simulink model "MMC_21_Level_Rectifier"  (R2023b)
settings: Solver=FixedStepAuto  StartTime=0.0  StopTime=0.5  RelTol=1e-3
libraries: spsSeriesRLCBranchLib x71, spsVoltageMeasurementLib x69, spsUniversalBridgeLib x60, spsCurrentMeasurementLib x8, slpidlib x7, spsRMSLib x3, spsACVoltageSourceLib x3, spsMeanLib x2, simulink x1, spsTHDLib x1, spspowerguiLib x1
(part 1 of 4)
settings Model: SimulationMode=accelerator  Creator=abc6820292  LastModifiedBy=Qu
settings SolverCC: ZeroCrossAlgorithm=Adaptive
settings DataIOCC: ReturnWorkspaceOutputs=off  Refine=10
settings DebuggingCC: IgnoredZcDiagnostic=none  UnconnectedInputMsg=warning  UnconnectedOutputMsg=warning  UnconnectedLineMsg=warning
settings ModelReferenceCC: EnableRefExpFcnMdlSchedulingChecks=on
settings RTWCC: DLArmComputeVersion=19.05

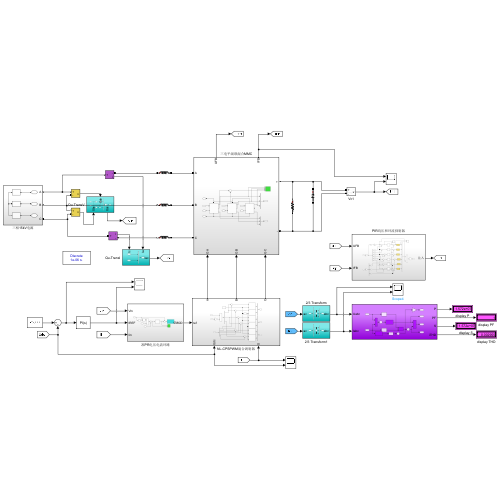
[thumbnail: Simulink's stored preview of the top-level diagram]
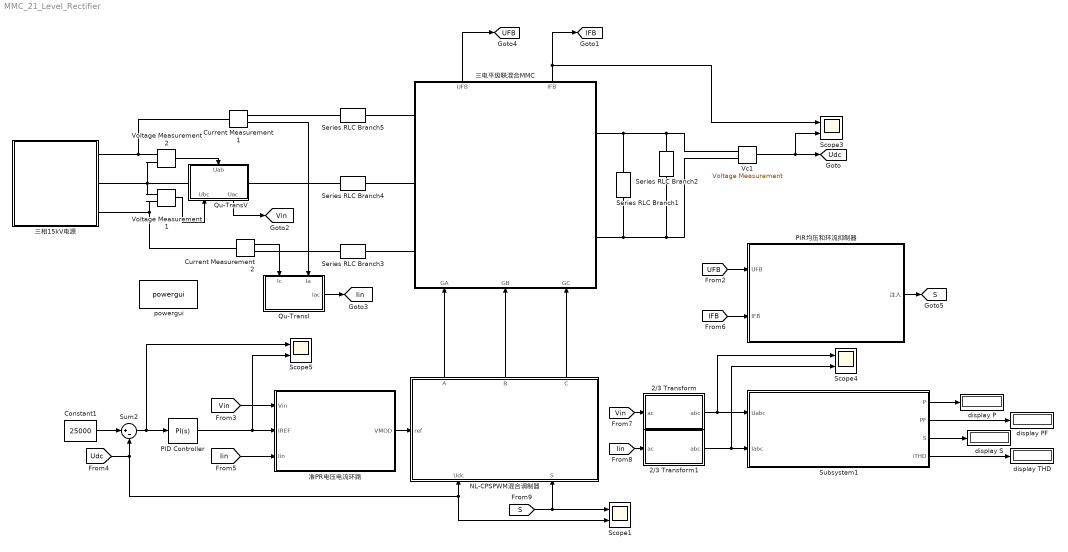
== system MMC_21_Level_Rectifier ==
  2/3 Transform : Subsystem
      settings: PortSchema="{\"entries\":[{\"content\":{\"sides\":[{\"content\":{},\"type\":\"ConnectorPlacement.EquallySpacedRectSide\",\"uuid\":\"58c40194-9a95-4e39-952e-f878bde7484e\"},{\"content\":{\"side\":\"RIGHT\"},\"type\":\"ConnectorPlacement.EquallySpacedRectSide\",\"uuid\":\"f51692e8-3ff2-4d72-808d-3667196a4526\"},{\"content\":{\"connectorIds\":[\"In1\"],\"side\":\"TOP\"},\"type\":\"ConnectorPlacement.EquallySpacedRectSide\",\"uuid\":\"0aab136b-5da5-45c4-8998-999ebe8b7f2f\"},{\"content\":{\"connectorIds\":[\"Out1\"],\"side\":\"BOTTOM\"},\"type\":\"ConnectorPlacement.EquallySpacedRectSide\",\"uuid\":\"32f5f4a5-4ebb-496b-828d-b973bd46b44e\"}]},\"type\":\"ConnectorPlacement.EquallySpacedConnector\",\"uuid\":\"3ef81af7-d426-47fb-88e3-e33e58eebb83\"}],\"packageUris\":[\"http://schema.mathworks.com/mf0/Connector/R2020b\"],\"version\":\"1.0\"}"
  2/3 Transform1 : Subsystem
      settings: PortSchema="{\"entries\":[{\"content\":{\"sides\":[{\"content\":{},\"type\":\"ConnectorPlacement.EquallySpacedRectSide\",\"uuid\":\"58c40194-9a95-4e39-952e-f878bde7484e\"},{\"content\":{\"side\":\"RIGHT\"},\"type\":\"ConnectorPlacement.EquallySpacedRectSide\",\"uuid\":\"f51692e8-3ff2-4d72-808d-3667196a4526\"},{\"content\":{\"connectorIds\":[\"In1\"],\"side\":\"TOP\"},\"type\":\"ConnectorPlacement.EquallySpacedRectSide\",\"uuid\":\"0aab136b-5da5-45c4-8998-999ebe8b7f2f\"},{\"content\":{\"connectorIds\":[\"Out1\"],\"side\":\"BOTTOM\"},\"type\":\"ConnectorPlacement.EquallySpacedRectSide\",\"uuid\":\"32f5f4a5-4ebb-496b-828d-b973bd46b44e\"}]},\"type\":\"ConnectorPlacement.EquallySpacedConnector\",\"uuid\":\"3ef81af7-d426-47fb-88e3-e33e58eebb83\"}],\"packageUris\":[\"http://schema.mathworks.com/mf0/Connector/R2020b\"],\"version\":\"1.0\"}"
  Constant1 : Constant  Value=25000
  Current Measurement1 : spsCurrentMeasurementLib/Current Measurement  PhasorSimulation=off  OutputType=Complex  PSBequivalent=0
  Current Measurement2 : spsCurrentMeasurementLib/Current Measurement  PhasorSimulation=off  OutputType=Complex  PSBequivalent=0
  NL-CPSPWM混合调制器 : Subsystem
      settings: PortSchema="{\"entries\":[{\"content\":{\"sides\":[{\"content\":{\"connectorIds\":[\"In1\"]},\"type\":\"ConnectorPlacement.EquallySpacedRectSide\",\"uuid\":\"86d8a801-af54-4615-919a-9a70996995f5\"},{\"content\":{\"side\":\"RIGHT\"},\"type\":\"ConnectorPlacement.EquallySpacedRectSide\",\"uuid\":\"9c099dd5-197a-4a29-8cd5-6822de601230\"},{\"content\":{\"connectorIds\":[\"Out1\",\"Out2\",\"Out3\"],\"side\":\"TOP\"},\"type\":\"ConnectorPlacement.EquallySpacedRectSide\",\"uuid\":\"5852d946-2383-4602-be71-32d16fa24bc3\"},{\"content\":{\"connectorIds\":[\"In2\",\"In3\"],\"side\":\"BOTTOM\"},\"type\":\"ConnectorPlacement.EquallySpacedRectSide\",\"uuid\":\"40763eea-52f3-43b7-92a8-ded335eb8a8b\"}]},\"type\":\"ConnectorPlacement.EquallySpacedConnector\",\"uuid\":\"a21c857f-e780-49b2-9a65-1676cf4540b1\"}],\"packageUris\":[\"http://schema.mathworks.com/mf0/Connector/R2020b\"],\"version\":\"1.0\"}"
  PID Controller : slpidlib/PID Controller  Controller=PI  Form=Parallel  TimeDomain=Continuous-time  UseExternalTs=off  SampleTime=-1  IntegratorMethod=Forward Euler  FilterMethod=Forward Euler  ControllerParametersSource=internal  P=0.12  I=6  UseKiTs=off  D=0  N=100  UseFilter=on  TunerSelectOption=Transfer Function Based (PID Tuner App)  InitialConditionSource=internal  InitialConditionForIntegrator=0  InitialConditionForFilter=0  DifferentiatorICPrevScaledInput=0  ExternalReset=none  TrackingMode=off  Kt=1  LimitOutput=off  SatLimitsSource=internal  UpperSaturationLimit=100  LowerSaturationLimit=-100  LinearizeAsGain=on  AntiWindupMode=none  Kb=1  LimitIntegrator=off  UpperIntegratorSaturationLimit=inf  LowerIntegratorSaturationLimit=-inf  POutMin=[]  POutMax=[]  IOutMin=[]  IOutMax=[]  DOutMin=[]  DOutMax=[]  NOutMin=[]  NOutMax=[]  SumOutMin=[]  SumOutMax=[]  SaturationOutMin=[]  SaturationOutMax=[]  PParamMin=[]  PParamMax=[]  IParamMin=[]  IParamMax=[]  DParamMin=[]  DParamMax=[]  NParamMin=[]  NParamMax=[]  KbParamMin=[]  KbParamMax=[]  KtParamMin=[]  KtParamMax=[]  KbOutMin=[]  KbOutMax=[]  KtOutMin=[]  KtOutMax=[]  IntegratorOutMin=[]  IntegratorOutMax=[]  FilterOutMin=[]  FilterOutMax=[]  SumI1OutMin=[]  SumI1OutMax=[]  SumI2OutMin=[]  SumI2OutMax=[]  SumI3OutMin=[]  SumI3OutMax=[]  SumI4OutMin=[]  SumI4OutMax=[]  SumDOutMin=[]  SumDOutMax=[]  DifferentiatorOutMin=[]  DifferentiatorOutMax=[]  FilterDiffOutCoefMin=[]  FilterDiffOutCoefMax=[]  ReciprocalOutMin=[]  ReciprocalOutMax=[]  SumDenOutMin=[]  SumDenOutMax=[]  SumNumOutMin=[]  SumNumOutMax=[]  DivideOutMin=[]  DivideOutMax=[]  UdiffTsProdOutMin=[]  UdiffTsProdOutMax=[]  NTsProdOutMin=[]  NTsProdOutMax=[]  UintegralTsProdOutMin=[]  UintegralTsProdOutMax=[]  UngainTsProdOutMin=[]  UngainTsProdOutMax=[]  ClampingZeroOutDataTypeStr=Inherit: Inherit via back propagation  ClampingZeroOutMin=[]  ClampingZeroOutMax=[]  FilterDenConstantOutDataTypeStr=Inherit: Inherit via back propagation  FilterDenConstantOutMin=[]  FilterDenConstantOutMax=[]  PCopyOutDataTypeStr=Inherit: Inherit via back propagation  PCopyOutMin=[]  PCopyOutMax=[]  NCopyOutDataTypeStr=Inherit: Inherit via back propagation  NCopyOutMin=[]  NCopyOutMax=[]  IntegratorContinuousStateAttributes=''  IntegratorStateMustResolveToSignalObject=off  IntegratorRTWStateStorageClass=Auto  FilterContinuousStateAttributes=''  FilterStateMustResolveToSignalObject=off  FilterRTWStateStorageClass=Auto  ParallelPVariant=InternalParameters  IdealPVariant=Disabled  IVariant=InternalParameters  DVariant=Disabled  IntegratorVariant=Continuous  SatVariant=Disabled  AWVariant=Passthrough  PCopyVariant=Disabled  TRVariant=Disabled  FdbkBlocksVariant=Forward  IdealPFdbkVariant=Disabled  SatFdbkVariant=Disabled  DerivativeFilterVariant=Disabled  NVariant=Disabled  NCopyVariant=Disabled_SignalSpec  FilterICVariant=Disabled  IntegratorICVariant=InternalICs  ExternalResetVariant=Disabled  TRSumVariant=Passthrough  SumFdbkVariant=Disabled  SumVariant=Sum_PI  TsampFilterVariant=InternalTs  TsampNgainVariant=Passthrough  TsampIntegralVariant=Disabled_SignalSpec  ExternalSaturationOutDataTypeStr=Inherit: Same as second input
  PIR均压和环流抑制器 : Subsystem
  Qu-TransI : Subsystem
      settings: PortSchema="{\"entries\":[{\"content\":{\"sides\":[{\"content\":{\"connectorIds\":[\"In1\",\"In2\"]},\"type\":\"ConnectorPlacement.EquallySpacedRectSide\",\"uuid\":\"58c40194-9a95-4e39-952e-f878bde7484e\"},{\"content\":{\"connectorIds\":[],\"side\":\"RIGHT\"},\"type\":\"ConnectorPlacement.EquallySpacedRectSide\",\"uuid\":\"f51692e8-3ff2-4d72-808d-3667196a4526\"},{\"content\":{\"connectorIds\":[],\"side\":\"TOP\"},\"type\":\"ConnectorPlacement.EquallySpacedRectSide\",\"uuid\":\"0aab136b-5da5-45c4-8998-999ebe8b7f2f\"},{\"content\":{\"connectorIds\":[\"Out1\"],\"side\":\"BOTTOM\"},\"type\":\"ConnectorPlacement.EquallySpacedRectSide\",\"uuid\":\"32f5f4a5-4ebb-496b-828d-b973bd46b44e\"}]},\"type\":\"ConnectorPlacement.EquallySpacedConnector\",\"uuid\":\"3ef81af7-d426-47fb-88e3-e33e58eebb83\"}],\"packageUris\":[\"http://schema.mathworks.com/mf0/Connector/R2020b\"],\"version\":\"1.0\"}"
  Qu-TransV : Subsystem
      settings: PortSchema="{\"entries\":[{\"content\":{\"sides\":[{\"content\":{\"connectorIds\":[\"In1\"]},\"type\":\"ConnectorPlacement.EquallySpacedRectSide\",\"uuid\":\"58c40194-9a95-4e39-952e-f878bde7484e\"},{\"content\":{\"connectorIds\":[\"In2\",\"Out1\"],\"side\":\"RIGHT\"},\"type\":\"ConnectorPlacement.EquallySpacedRectSide\",\"uuid\":\"f51692e8-3ff2-4d72-808d-3667196a4526\"},{\"content\":{\"side\":\"TOP\"},\"type\":\"ConnectorPlacement.EquallySpacedRectSide\",\"uuid\":\"0aab136b-5da5-45c4-8998-999ebe8b7f2f\"},{\"content\":{\"side\":\"BOTTOM\"},\"type\":\"ConnectorPlacement.EquallySpacedRectSide\",\"uuid\":\"185ce796-68e2-4136-8080-97dc86d2ba54\"}]},\"type\":\"ConnectorPlacement.EquallySpacedConnector\",\"uuid\":\"3ef81af7-d426-47fb-88e3-e33e58eebb83\"}],\"packageUris\":[\"http://schema.mathworks.com/mf0/Connector/R2020b\"],\"version\":\"1.0\"}"
  Scope{1,3..5} (4 alike) : Scope  NumInputPorts=2
  Series RLC Branch1 : spsSeriesRLCBranchLib/Series RLC Branch  LConnTagsString=__new0  RConnTagsString=__new0  BranchType=R  Resistance=40  Inductance=6e-4  SetiL0=off  InitialCurrent=0  Capacitance=1e-6  Setx0=off  InitialVoltage=0  Measurements=None
  Series RLC Branch2 : spsSeriesRLCBranchLib/Series RLC Branch  LConnTagsString=__new0  RConnTagsString=__new0  BranchType=C  Resistance=25  Inductance=6e-4  SetiL0=off  InitialCurrent=0  Capacitance=2e-3  Setx0=on  InitialVoltage=23000  Measurements=None
  Series RLC Branch3 : spsSeriesRLCBranchLib/Series RLC Branch  LConnTagsString=__new0  RConnTagsString=__new0  BranchType=L  Resistance=25  Inductance=1e-3  SetiL0=off  InitialCurrent=0  Capacitance=1e-6  Setx0=off  InitialVoltage=0  Measurements=None
  Series RLC Branch4 : spsSeriesRLCBranchLib/Series RLC Branch  LConnTagsString=__new0  RConnTagsString=__new0  BranchType=L  Resistance=25  Inductance=1e-3  SetiL0=off  InitialCurrent=0  Capacitance=1e-6  Setx0=off  InitialVoltage=0  Measurements=None
  Series RLC Branch5 : spsSeriesRLCBranchLib/Series RLC Branch  LConnTagsString=__new0  RConnTagsString=__new0  BranchType=L  Resistance=25  Inductance=1e-3  SetiL0=off  InitialCurrent=0  Capacitance=1e-6  Setx0=off  InitialVoltage=0  Measurements=None
  Subsystem1 : Subsystem
  Sum2 : Sum  Inputs=|+-
  Vc1 : spsVoltageMeasurementLib/Voltage Measurement  PhasorSimulation=off  OutputType=Complex  PSBequivalent=0
  Voltage Measurement1 : spsVoltageMeasurementLib/Voltage Measurement  PhasorSimulation=off  OutputType=Complex  PSBequivalent=0
  Voltage Measurement2 : spsVoltageMeasurementLib/Voltage Measurement  PhasorSimulation=off  OutputType=Complex  PSBequivalent=0
  display P : Display
  display PF : Display
  display S : Display
  display THD : Display
  powergui : spspowerguiLib/powergui  Priority=1  SimulationMode=Discrete  SampleTime=1e-6  frequency=60  Iterations=50  frequencyindice=50  Pbase=100e6  ErrMax=1e-4  UnitsV=kV  UnitsW=MW  buscounter=0  FunctionMessages=off  echomessages=off  EnableUseOfTLC=off  CurrentSourceSwitches=off  DisableSnubberDevices=off  DisableRonSwitches=off  DisableVfSwitches=off  DisplayEquations=off  AutomaticDiscreteSolvers=off  SolverType=Tustin/Backward Euler (TBE)  Interpol=off  ExternalGateDelay=off  methode=off  Ts=100  x0status=blocks  SPID=on  SwTol=0  HookPort=off  NonlinearTolerance=1e-4  nMaxIteration=100  ContinueOnMaxIteration=off  RestoreLinks=warning  ResistiveCurrentMeasurement=off  Frange=[0:2:500]  Ylog=off  Xlog=on  ShowGrid=off  save=off  variable=ZData  structure=0  ZoomFFT=off  StartTime=0.0  cycles=1  DisplayStyle=1  fundamental=60  FreqAxis=off  MaxFrequency=1000  frequencyindicesteady=1  RmsSteady=1  display=off
  三电平级联混合MMC : Subsystem
      settings: PortSchema="{\"entries\":[{\"content\":{\"sides\":[{\"content\":{\"connectorIds\":[\"LConn1\",\"LConn2\",\"LConn3\"]},\"type\":\"ConnectorPlacement.EquallySpacedRectSide\",\"uuid\":\"b14efc91-6835-4ed7-8c1d-e2670cf7c179\"},{\"content\":{\"connectorIds\":[\"RConn1\",\"RConn2\"],\"side\":\"RIGHT\"},\"type\":\"ConnectorPlacement.EquallySpacedRectSide\",\"uuid\":\"133f26b8-b252-4d3c-80df-0b09760e0c14\"},{\"content\":{\"connectorIds\":[\"Out1\",\"Out2\"],\"side\":\"TOP\"},\"type\":\"ConnectorPlacement.EquallySpacedRectSide\",\"uuid\":\"c058e102-7791-48c2-b9e4-e80cedcfd34e\"},{\"content\":{\"connectorIds\":[\"In1\",\"In2\",\"In3\"],\"side\":\"BOTTOM\"},\"type\":\"ConnectorPlacement.EquallySpacedRectSide\",\"uuid\":\"7bcd8845-3331-4b31-8039-611891643c20\"}]},\"type\":\"ConnectorPlacement.EquallySpacedConnector\",\"uuid\":\"173e4324-58a1-473c-9df3-d0606e4a673f\"}],\"packageUris\":[\"http://schema.mathworks.com/mf0/Connector/R2020b\"],\"version\":\"1.0\"}"
  三相15kV电源 : Subsystem
  准PR电压电流环路 : Subsystem
  tag scope: IFB=global, Iin=global, S=global, UFB=global, Udc=global, Vin=global
  wires:
  Voltage Measurement1/1 -> Qu-TransV/2(Ubc)
  Subsystem1/1(P) -> display P/1
  2/3 Transform/1(abc) -> Subsystem1/1(Uabc), Scope4/1
  [Iin] -> 2/3 Transform1/1(ac)
  Qu-TransI/1(Iac) -> [Iin]
  Voltage Measurement2/1 -> Qu-TransV/1(Uab)
  Subsystem1/4(iTHD) -> display THD/1
  [Vin] -> 准PR电压电流环路/1(Vin)
  [Iin] -> 准PR电压电流环路/3(Iin)
  准PR电压电流环路/1(VMOD) -> NL-CPSPWM混合调制器/1(ref)
  Subsystem1/2(PF) -> display PF/1
  Current Measurement2/1 -> Qu-TransI/1(Ic)
  Sum2/1 -> Scope5/1, PID Controller/1
  Qu-TransV/1(Uac) -> [Vin]
  Subsystem1/3(S) -> display S/1
  [Vin] -> 2/3 Transform/1(ac)
  Current Measurement1/1 -> Qu-TransI/2(Ia)
  2/3 Transform1/1(abc) -> Subsystem1/2(Iabc), Scope4/2
  Vc1/1 -> [Udc], Scope3/2
  三电平级联混合MMC/2(IFB) -> [IFB], Scope3/1
  三电平级联混合MMC/1(UFB) -> [UFB]
  [UFB] -> PIR均压和环流抑制器/1(UFB)
  [IFB] -> PIR均压和环流抑制器/2(IFB)
  [S] -> NL-CPSPWM混合调制器/3(S), Scope1/1
  [Udc] -> NL-CPSPWM混合调制器/2(Udc), Scope1/2, Sum2/2
  Constant1/1 -> Sum2/1
  PIR均压和环流抑制器/1(注入) -> [S]
  PID Controller/1 -> Scope5/2, 准PR电压电流环路/2(IREF)
  NL-CPSPWM混合调制器/1(A) -> 三电平级联混合MMC/1(GA)
  NL-CPSPWM混合调制器/2(B) -> 三电平级联混合MMC/2(GB)
  NL-CPSPWM混合调制器/3(C) -> 三电平级联混合MMC/3(GC)
  connections:
  Voltage Measurement2/LConn1 -- 三相15kV电源/RConn1 -- Current Measurement1/LConn1
  Voltage Measurement1/LConn2 -- 三相15kV电源/RConn3 -- Current Measurement2/LConn1
  Voltage Measurement1/LConn1 -- Voltage Measurement2/LConn2 -- Series RLC Branch4/LConn1 -- 三相15kV电源/RConn2
  Vc1/LConn1 -- Series RLC Branch2/LConn1 -- Series RLC Branch1/LConn1 -- 三电平级联混合MMC/RConn1
  Series RLC Branch5/LConn1 -- Current Measurement1/RConn1
  Vc1/LConn2 -- Series RLC Branch2/RConn1 -- Series RLC Branch1/RConn1 -- 三电平级联混合MMC/RConn2
  Series RLC Branch3/RConn1 -- 三电平级联混合MMC/LConn3
  Series RLC Branch3/LConn1 -- Current Measurement2/RConn1
  Series RLC Branch4/RConn1 -- 三电平级联混合MMC/LConn2
  Series RLC Branch5/RConn1 -- 三电平级联混合MMC/LConn1

== system MMC_21_Level_Rectifier/2//3 Transform ==
  ac : Inport
  Demux : Demux  Outputs=2
  Mux : Mux  Inputs=3
  Sum1 : Sum  Inputs=-|-
  abc : Outport
  wires:
  Sum1/1 -> Mux/2
  Mux/1 -> abc/1
  Demux/1 -> Sum1/1, Mux/1
  ac/1 -> Demux/1
  Demux/2 -> Sum1/2, Mux/3

== system MMC_21_Level_Rectifier/2//3 Transform1 ==
  ac : Inport
  Demux : Demux  Outputs=2
  Mux : Mux  Inputs=3
  Sum1 : Sum  Inputs=-|-
  abc : Outport
  wires:
  Sum1/1 -> Mux/2
  Mux/1 -> abc/1
  Demux/1 -> Sum1/1, Mux/1
  ac/1 -> Demux/1
  Demux/2 -> Sum1/2, Mux/3

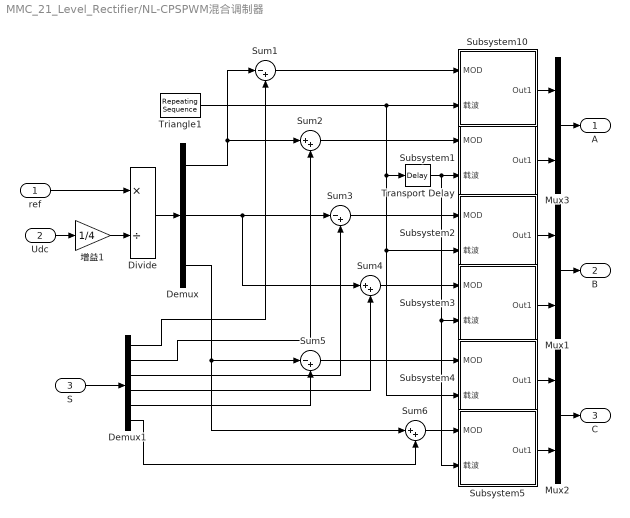
== system MMC_21_Level_Rectifier/NL-CPSPWM混合调制器 ==
  ref : Inport
  Udc : Inport  Port=2
  S : Inport  Port=3
  Demux : Demux  Outputs=3
  Demux1 : Demux  Outputs=6
  Divide : Product  Inputs=*/
  Mux1 : Mux  Inputs=2
  Mux2 : Mux  Inputs=2
  Mux3 : Mux  Inputs=2
  Subsystem1 : Subsystem
  Subsystem10 : Subsystem
  Subsystem2 : Subsystem
  Subsystem3 : Subsystem
  Subsystem4 : Subsystem
  Subsystem5 : Subsystem
  Sum1 : Sum  Inputs=|-+
  Sum2 : Sum  Inputs=|++
  Sum3 : Sum  Inputs=|-+
  Sum4 : Sum  Inputs=|++
  Sum5 : Sum  Inputs=|-+
  Sum6 : Sum  Inputs=|++
  Transport Delay : TransportDelay  DelayTime=1/800/4
  Triangle1 : simulink/Sources/Repeating Sequence  rep_seq_t=[0 1/800/2 1/800]  rep_seq_y=[-1 1 -1]
  增益1 : Gain  Gain=1/4
  A : Outport
  B : Outport  Port=2
  C : Outport  Port=3
  wires:
  ref/1 -> Divide/1
  增益1/1 -> Divide/2
  Udc/1 -> 增益1/1
  Triangle1/1 -> Subsystem4/2(载波), Subsystem2/2(载波), Transport Delay/1, Subsystem10/2(载波)
  Divide/1 -> Demux/1
  Mux3/1 -> A/1
  Subsystem10/1(Out1) -> Mux3/1
  Subsystem1/1(Out1) -> Mux3/2
  Subsystem3/1(Out1) -> Mux1/2
  Subsystem2/1(Out1) -> Mux1/1
  Mux1/1 -> B/1
  Mux2/1 -> C/1
  Subsystem4/1(Out1) -> Mux2/1
  Subsystem5/1(Out1) -> Mux2/2
  Transport Delay/1 -> Subsystem1/2(载波), Subsystem5/2(载波), Subsystem3/2(载波)
  Sum4/1 -> Subsystem3/1(MOD)
  S/1 -> Demux1/1
  Sum1/1 -> Subsystem10/1(MOD)
  Sum2/1 -> Subsystem1/1(MOD)
  Demux/1 -> Sum2/1, Sum1/1
  Demux/2 -> Sum4/1, Sum3/1
  Sum6/1 -> Subsystem5/1(MOD)
  Sum5/1 -> Subsystem4/1(MOD)
  Demux/3 -> Sum6/1, Sum5/1
  Sum3/1 -> Subsystem2/1(MOD)
  Demux1/6 -> Sum6/2
  Demux1/5 -> Sum5/2
  Demux1/4 -> Sum4/2
  Demux1/3 -> Sum3/2
  Demux1/2 -> Sum2/2
  Demux1/1 -> Sum1/2

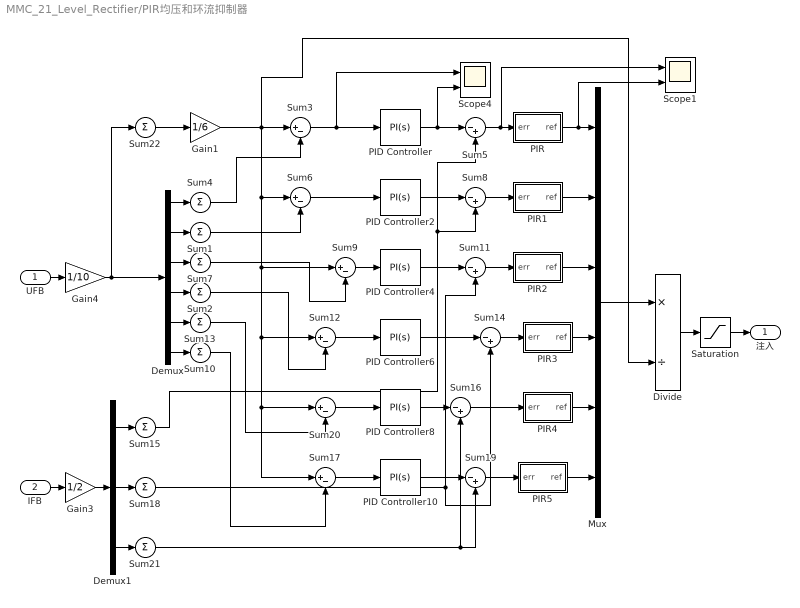
== system MMC_21_Level_Rectifier/PIR均压和环流抑制器 ==
  UFB : Inport
  IFB : Inport  Port=2
  Demux : Demux  Outputs=6
  Demux1 : Demux  Outputs=3
  Divide : Product  Inputs=*/
  Gain1 : Gain  Gain=1/6
  Gain3 : Gain  Gain=1/2
  Gain4 : Gain  Gain=1/10
  Mux : Mux  Inputs=6
  PID Controller{,2,4,6,8,10} (6 alike) : slpidlib/PID Controller  Controller=PI  Form=Parallel  TimeDomain=Continuous-time  UseExternalTs=off  SampleTime=-1  IntegratorMethod=Forward Euler  FilterMethod=Forward Euler  ControllerParametersSource=internal  P=0.02  I=2.35  UseKiTs=off  D=0  N=100  UseFilter=on  TunerSelectOption=Transfer Function Based (PID Tuner App)  InitialConditionSource=internal  InitialConditionForIntegrator=0  InitialConditionForFilter=0  DifferentiatorICPrevScaledInput=0  ExternalReset=none  TrackingMode=off  Kt=1  LimitOutput=off  SatLimitsSource=internal  UpperSaturationLimit=inf  LowerSaturationLimit=-inf  LinearizeAsGain=on  AntiWindupMode=none  Kb=1  LimitIntegrator=off  UpperIntegratorSaturationLimit=inf  LowerIntegratorSaturationLimit=-inf  POutMin=[]  POutMax=[]  IOutMin=[]  IOutMax=[]  DOutMin=[]  DOutMax=[]  NOutMin=[]  NOutMax=[]  SumOutMin=[]  SumOutMax=[]  SaturationOutMin=[]  SaturationOutMax=[]  PParamMin=[]  PParamMax=[]  IParamMin=[]  IParamMax=[]  DParamMin=[]  DParamMax=[]  NParamMin=[]  NParamMax=[]  KbParamMin=[]  KbParamMax=[]  KtParamMin=[]  KtParamMax=[]  KbOutMin=[]  KbOutMax=[]  KtOutMin=[]  KtOutMax=[]  IntegratorOutMin=[]  IntegratorOutMax=[]  FilterOutMin=[]  FilterOutMax=[]  SumI1OutMin=[]  SumI1OutMax=[]  SumI2OutMin=[]  SumI2OutMax=[]  SumI3OutMin=[]  SumI3OutMax=[]  SumI4OutMin=[]  SumI4OutMax=[]  SumDOutMin=[]  SumDOutMax=[]  DifferentiatorOutMin=[]  DifferentiatorOutMax=[]  FilterDiffOutCoefMin=[]  FilterDiffOutCoefMax=[]  ReciprocalOutMin=[]  ReciprocalOutMax=[]  SumDenOutMin=[]  SumDenOutMax=[]  SumNumOutMin=[]  SumNumOutMax=[]  DivideOutMin=[]  DivideOutMax=[]  UdiffTsProdOutMin=[]  UdiffTsProdOutMax=[]  NTsProdOutMin=[]  NTsProdOutMax=[]  UintegralTsProdOutMin=[]  UintegralTsProdOutMax=[]  UngainTsProdOutMin=[]  UngainTsProdOutMax=[]  ClampingZeroOutDataTypeStr=Inherit: Inherit via back propagation  ClampingZeroOutMin=[]  ClampingZeroOutMax=[]  FilterDenConstantOutDataTypeStr=Inherit: Inherit via back propagation  FilterDenConstantOutMin=[]  FilterDenConstantOutMax=[]  PCopyOutDataTypeStr=Inherit: Inherit via back propagation  PCopyOutMin=[]  PCopyOutMax=[]  NCopyOutDataTypeStr=Inherit: Inherit via back propagation  NCopyOutMin=[]  NCopyOutMax=[]  IntegratorContinuousStateAttributes=''  IntegratorStateMustResolveToSignalObject=off  IntegratorRTWStateStorageClass=Auto  FilterContinuousStateAttributes=''  FilterStateMustResolveToSignalObject=off  FilterRTWStateStorageClass=Auto  ParallelPVariant=InternalParameters  IdealPVariant=Disabled  IVariant=InternalParameters  DVariant=Disabled  IntegratorVariant=Continuous  SatVariant=Disabled  AWVariant=Passthrough  PCopyVariant=Disabled  TRVariant=Disabled  FdbkBlocksVariant=Forward  IdealPFdbkVariant=Disabled  SatFdbkVariant=Disabled  DerivativeFilterVariant=Disabled  NVariant=Disabled  NCopyVariant=Disabled_SignalSpec  FilterICVariant=Disabled  IntegratorICVariant=InternalICs  ExternalResetVariant=Disabled  TRSumVariant=Passthrough  SumFdbkVariant=Disabled  SumVariant=Sum_PI  TsampFilterVariant=InternalTs  TsampNgainVariant=Passthrough  TsampIntegralVariant=Disabled_SignalSpec  ExternalSaturationOutDataTypeStr=Inherit: Same as second input
  PIR : Subsystem  TreatAsAtomicUnit=on  mask{Kp=1, Kr=10, Wc=5, Upper=4000, Lower=-4000}
  PIR1 : Subsystem  TreatAsAtomicUnit=on  mask{Kp=1, Kr=10, Wc=5, Upper=4000, Lower=-4000}
  PIR2 : Subsystem  TreatAsAtomicUnit=on  mask{Kp=1, Kr=10, Wc=5, Upper=4000, Lower=-4000}
  PIR3 : Subsystem  TreatAsAtomicUnit=on  mask{Kp=1, Kr=10, Wc=5, Upper=4000, Lower=-4000}
  PIR4 : Subsystem  TreatAsAtomicUnit=on  mask{Kp=1, Kr=10, Wc=5, Upper=4000, Lower=-4000}
  PIR5 : Subsystem  TreatAsAtomicUnit=on  mask{Kp=1, Kr=10, Wc=5, Upper=400, Lower=-400}
  Saturation : Saturate  UpperLimit=1  LowerLimit=-1
  Scope1 : Scope  NumInputPorts=2
  Scope4 : Scope  NumInputPorts=2
  Sum{1..2,4,7,10,13,15,18,21..22} (10 alike) : Sum  Inputs=+
  Sum{5,8,11,14,16,19} (6 alike) : Sum  Inputs=|-+
  Sum{3,6,9,12,17,20} (6 alike) : Sum  Inputs=|+-
  注入 : Outport  VectorParamsAs1DForOutWhenUnconnected=off
  wires:
  PID Controller4/1 -> Sum11/1
  Sum4/1 -> Sum3/2
  Gain1/1 -> Divide/2, Sum17/1, Sum20/1, Sum12/1, Sum9/1, Sum6/1, Sum3/1
  Sum14/1 -> PIR3/1(err)
  PID Controller8/1 -> Sum16/1
  Sum21/1 -> Sum19/2, Sum16/2
  Sum12/1 -> PID Controller6/1
  Sum8/1 -> PIR1/1(err)
  Sum15/1 -> Sum8/2, Sum5/2
  Sum10/1 -> Sum17/2
  PID Controller6/1 -> Sum14/1
  Sum9/1 -> PID Controller4/1
  Sum11/1 -> PIR2/1(err)
  Sum2/1 -> Sum12/2
  Sum20/1 -> PID Controller8/1
  Sum18/1 -> Sum11/2, Sum14/2
  PID Controller/1 -> Scope4/2, Sum5/1
  Sum16/1 -> PIR4/1(err)
  Sum7/1 -> Sum9/2
  Sum19/1 -> PIR5/1(err)
  Sum6/1 -> PID Controller2/1
  PID Controller10/1 -> Sum19/1
  Sum17/1 -> PID Controller10/1
  PID Controller2/1 -> Sum8/1
  Sum13/1 -> Sum20/2
  Sum5/1 -> Scope1/1, PIR/1(err)
  Sum3/1 -> Scope4/1, PID Controller/1
  Saturation/1 -> 注入/1
  Demux/1 -> Sum4/1
  Demux/2 -> Sum1/1
  Demux/3 -> Sum7/1
  Demux/4 -> Sum2/1
  Demux/5 -> Sum13/1
  Demux/6 -> Sum10/1
  Sum1/1 -> Sum6/2
  UFB/1 -> Gain4/1
  IFB/1 -> Gain3/1
  Gain3/1 -> Demux1/1
  Demux1/1 -> Sum15/1
  Demux1/2 -> Sum18/1
  Demux1/3 -> Sum21/1
  PIR/1(ref) -> Scope1/2, Mux/1
  PIR1/1(ref) -> Mux/2
  PIR2/1(ref) -> Mux/3
  PIR3/1(ref) -> Mux/4
  PIR4/1(ref) -> Mux/5
  PIR5/1(ref) -> Mux/6
  Mux/1 -> Divide/1
  Gain4/1 -> Sum22/1, Demux/1
  Sum22/1 -> Gain1/1
  Divide/1 -> Saturation/1

== system MMC_21_Level_Rectifier/Qu-TransI ==
  Ic : Inport
  Ia : Inport  Port=2
  Mux : Mux  Inputs=2
  Iac : Outport
  wires:
  Ia/1 -> Mux/1
  Mux/1 -> Iac/1
  Ic/1 -> Mux/2

== system MMC_21_Level_Rectifier/Qu-TransV ==
  Uab : Inport
  Ubc : Inport  Port=2
  Gain2 : Gain  Gain=1/3
  Gain3 : Gain  Gain=2
  Gain4 : Gain  Gain=2
  Mux : Mux  Inputs=2
  Sum2 : Sum  Inputs=--|
  Sum6 : Sum  Inputs=|++
  Uac : Outport
  wires:
  Uab/1 -> Sum2/1, Gain4/1
  Gain4/1 -> Sum6/1
  Ubc/1 -> Gain3/1, Sum6/2
  Sum2/1 -> Mux/2
  Sum6/1 -> Mux/1
  Gain3/1 -> Sum2/2
  Mux/1 -> Gain2/1
  Gain2/1 -> Uac/1

== system MMC_21_Level_Rectifier/Subsystem1 ==
  Uabc : Inport
  Iabc : Inport  Port=2
  Divide2 : Product  Inputs=*/
  Gain6 : Gain  Gain=1/3
  Mean : spsMeanLib/Mean  Freq=100  Vinit=0  Ts=0
  Mean1 : spsMeanLib/Mean  Freq=20000  Vinit=0  Ts=0
  Product2 : Product
  Product4 : Product
  RMS2 : spsRMSLib/RMS  TrueRMS=on  Freq=50  RMSInit=0  Ts=0
  RMS3 : spsRMSLib/RMS  TrueRMS=on  Freq=50  RMSInit=0  Ts=0
  Sum1 : Sum  Inputs=+
  Sum6 : Sum  Inputs=+
  Sum7 : Sum  Inputs=+
  THD : spsTHDLib/THD  Freq=50  Ts=0
  P : Outport
  PF : Outport  Port=2
  S : Outport  Port=3
  iTHD : Outport  Port=4
  wires:
  Mean1/1 -> THD/1
  THD/1 -> Sum1/1
  Iabc/1 -> RMS2/1, Product2/2, Mean1/1
  Mean/1 -> Divide2/1, P/1
  Sum7/1 -> Divide2/2, S/1
  Uabc/1 -> Product2/1, RMS3/1
  Gain6/1 -> iTHD/1
  Sum1/1 -> Gain6/1
  RMS2/1 -> Product4/2
  Divide2/1 -> PF/1
  Product2/1 -> Sum6/1
  Sum6/1 -> Mean/1
  Product4/1 -> Sum7/1
  RMS3/1 -> Product4/1

== system MMC_21_Level_Rectifier/三电平级联混合MMC ==
  GA : Inport
  GB : Inport  Port=2
  GC : Inport  Port=3
  Mux : Mux  Inputs=3
  Mux1 : Mux  Inputs=3
  Scope12 : Scope  NumInputPorts=4
  Subsystem1 : Subsystem
      settings: PortSchema="{\"entries\":[{\"content\":{\"sides\":[{\"content\":{\"connectorIds\":[\"In1\",\"LConn1\"]},\"type\":\"ConnectorPlacement.EquallySpacedRectSide\",\"uuid\":\"42b8d19e-8d66-4598-9931-1794559657ef\"},{\"content\":{\"connectorIds\":[\"Out1\",\"Out2\",\"Out3\"],\"side\":\"RIGHT\"},\"type\":\"ConnectorPlacement.EquallySpacedRectSide\",\"uuid\":\"f40691a8-1dc9-415e-92e1-8ab81841390a\"},{\"content\":{\"connectorIds\":[\"LConn2\"],\"side\":\"TOP\"},\"type\":\"ConnectorPlacement.EquallySpacedRectSide\",\"uuid\":\"2eee6a4a-e939-4f77-b73a-57c25ce7275b\"},{\"content\":{\"connectorIds\":[\"RConn1\"],\"side\":\"BOTTOM\"},\"type\":\"ConnectorPlacement.EquallySpacedRectSide\",\"uuid\":\"ef7847eb-cc02-4736-bf04-c09726753cc8\"}]},\"type\":\"ConnectorPlacement.EquallySpacedConnector\",\"uuid\":\"4781621e-30e8-40f4-8fb9-337a1adad445\"}],\"packageUris\":[\"http://schema.mathworks.com/mf0/Connector/R2020b\"],\"version\":\"1.0\"}"
  Subsystem2 : Subsystem
      settings: PortSchema="{\"entries\":[{\"content\":{\"sides\":[{\"content\":{\"connectorIds\":[\"In1\",\"LConn1\"]},\"type\":\"ConnectorPlacement.EquallySpacedRectSide\",\"uuid\":\"42b8d19e-8d66-4598-9931-1794559657ef\"},{\"content\":{\"connectorIds\":[\"Out1\",\"Out2\",\"Out3\"],\"side\":\"RIGHT\"},\"type\":\"ConnectorPlacement.EquallySpacedRectSide\",\"uuid\":\"f40691a8-1dc9-415e-92e1-8ab81841390a\"},{\"content\":{\"connectorIds\":[\"LConn2\"],\"side\":\"TOP\"},\"type\":\"ConnectorPlacement.EquallySpacedRectSide\",\"uuid\":\"2eee6a4a-e939-4f77-b73a-57c25ce7275b\"},{\"content\":{\"connectorIds\":[\"RConn1\"],\"side\":\"BOTTOM\"},\"type\":\"ConnectorPlacement.EquallySpacedRectSide\",\"uuid\":\"ef7847eb-cc02-4736-bf04-c09726753cc8\"}]},\"type\":\"ConnectorPlacement.EquallySpacedConnector\",\"uuid\":\"4781621e-30e8-40f4-8fb9-337a1adad445\"}],\"packageUris\":[\"http://schema.mathworks.com/mf0/Connector/R2020b\"],\"version\":\"1.0\"}"
  Subsystem3 : Subsystem
      settings: PortSchema="{\"entries\":[{\"content\":{\"sides\":[{\"content\":{\"connectorIds\":[\"In1\",\"LConn1\"]},\"type\":\"ConnectorPlacement.EquallySpacedRectSide\",\"uuid\":\"42b8d19e-8d66-4598-9931-1794559657ef\"},{\"content\":{\"connectorIds\":[\"Out1\",\"Out2\",\"Out3\"],\"side\":\"RIGHT\"},\"type\":\"ConnectorPlacement.EquallySpacedRectSide\",\"uuid\":\"f40691a8-1dc9-415e-92e1-8ab81841390a\"},{\"content\":{\"connectorIds\":[\"LConn2\"],\"side\":\"TOP\"},\"type\":\"ConnectorPlacement.EquallySpacedRectSide\",\"uuid\":\"2eee6a4a-e939-4f77-b73a-57c25ce7275b\"},{\"content\":{\"connectorIds\":[\"RConn1\"],\"side\":\"BOTTOM\"},\"type\":\"ConnectorPlacement.EquallySpacedRectSide\",\"uuid\":\"ef7847eb-cc02-4736-bf04-c09726753cc8\"}]},\"type\":\"ConnectorPlacement.EquallySpacedConnector\",\"uuid\":\"4781621e-30e8-40f4-8fb9-337a1adad445\"}],\"packageUris\":[\"http://schema.mathworks.com/mf0/Connector/R2020b\"],\"version\":\"1.0\"}"
  Sum : Sum  Inputs=|+-
  A : PMIOPort  Side=Left
  B : PMIOPort  Port=2  Side=Left
  C : PMIOPort  Port=3  Side=Left
  + : PMIOPort  Port=4  Side=Right
  - : PMIOPort  Port=5  Side=Right
  UFB : Outport
  IFB : Outport  Port=2
  wires:
  Mux/1 -> UFB/1
  Mux1/1 -> IFB/1
  Subsystem2/1(Uc) -> Scope12/1, Mux/1
  Subsystem1/1(Uc) -> Scope12/2, Mux/2
  Subsystem2/3(I) -> Mux1/1
  Subsystem1/3(I) -> Mux1/2
  GA/1 -> Subsystem2/1(GA)
  GB/1 -> Subsystem1/1(GA)
  GC/1 -> Subsystem3/1(GA)
  Subsystem3/3(I) -> Mux1/3
  Subsystem3/1(Uc) -> Mux/3, Scope12/3
  Subsystem2/2(Uac) -> Sum/1
  Subsystem1/2(Uac) -> Sum/2
  Sum/1 -> Scope12/4
  connections:
  A/RConn1 -- Subsystem2/LConn1
  +/RConn1 -- Subsystem3/LConn2 -- Subsystem1/LConn2 -- Subsystem2/LConn2
  Subsystem2/RConn1 -- Subsystem3/RConn1 -- Subsystem1/RConn1 -- -/RConn1
  Subsystem1/LConn1 -- B/RConn1
  Subsystem3/LConn1 -- C/RConn1

== system MMC_21_Level_Rectifier/三相15kV电源 ==
  AC Voltage Source : spsACVoltageSourceLib/AC Voltage Source  Amplitude=12000  Phase=0  Frequency=50  SampleTime=0  Measurements=None  BusType=swing  Pref=10e3  Qref=0  Qmin=-inf  Qmax=+inf
  AC Voltage Source1 : spsACVoltageSourceLib/AC Voltage Source  Amplitude=12000  Phase=120  Frequency=50  SampleTime=0  Measurements=None  BusType=swing  Pref=10e3  Qref=0  Qmin=-inf  Qmax=+inf
  AC Voltage Source2 : spsACVoltageSourceLib/AC Voltage Source  Amplitude=12000  Phase=-120  Frequency=50  SampleTime=0  Measurements=None  BusType=swing  Pref=10e3  Qref=0  Qmin=-inf  Qmax=+inf
  A : PMIOPort  Side=Right
  B : PMIOPort  Port=2  Side=Right
  C : PMIOPort  Port=3  Side=Right
  connections:
  AC Voltage Source2/RConn1 -- C/RConn1
  A/RConn1 -- AC Voltage Source/RConn1
  B/RConn1 -- AC Voltage Source1/RConn1
  AC Voltage Source/LConn1 -- AC Voltage Source2/LConn1 -- AC Voltage Source1/LConn1

== system MMC_21_Level_Rectifier/准PR电压电流环路 ==
  Vin : Inport
  IREF : Inport  Port=2
  Iin : Inport  Port=3
  2/3 Transform : Subsystem
      settings: PortSchema="{\"entries\":[{\"content\":{\"sides\":[{\"content\":{},\"type\":\"ConnectorPlacement.EquallySpacedRectSide\",\"uuid\":\"58c40194-9a95-4e39-952e-f878bde7484e\"},{\"content\":{\"side\":\"RIGHT\"},\"type\":\"ConnectorPlacement.EquallySpacedRectSide\",\"uuid\":\"f51692e8-3ff2-4d72-808d-3667196a4526\"},{\"content\":{\"connectorIds\":[\"In1\"],\"side\":\"TOP\"},\"type\":\"ConnectorPlacement.EquallySpacedRectSide\",\"uuid\":\"0aab136b-5da5-45c4-8998-999ebe8b7f2f\"},{\"content\":{\"connectorIds\":[\"Out1\"],\"side\":\"BOTTOM\"},\"type\":\"ConnectorPlacement.EquallySpacedRectSide\",\"uuid\":\"32f5f4a5-4ebb-496b-828d-b973bd46b44e\"}]},\"type\":\"ConnectorPlacement.EquallySpacedConnector\",\"uuid\":\"3ef81af7-d426-47fb-88e3-e33e58eebb83\"}],\"packageUris\":[\"http://schema.mathworks.com/mf0/Connector/R2020b\"],\"version\":\"1.0\"}"
  Digital PR A-C : Subsystem  mask{Kp=10, Kr=1000, Wc=5, Ts=1/32000, Upper=25000, Lower=-25000}
      mask DialogControl ParameterGroupVar Prompt: 参数
  Divide : Product  Inputs=*/
  Product2 : Product
  RMS : spsRMSLib/RMS  TrueRMS=on  Freq=50  RMSInit=8000  Ts=0
  Scope6 : Scope  NumInputPorts=2
  Sum5 : Sum  Inputs=+-|
  Sum6 : Sum  Inputs=|+-
  VMOD : Outport
  wires:
  IREF/1 -> Product2/2
  Sum6/1 -> Digital PR A-C/1(err), Scope6/2
  Iin/1 -> Sum6/2
  Digital PR A-C/1(out) -> Scope6/1, Sum5/2
  Sum5/1 -> 2/3 Transform/1(ac)
  2/3 Transform/1(abc) -> VMOD/1
  Product2/1 -> Sum6/1
  Divide/1 -> Product2/1
  Vin/1 -> RMS/1, Divide/1, Sum5/1
  RMS/1 -> Divide/2

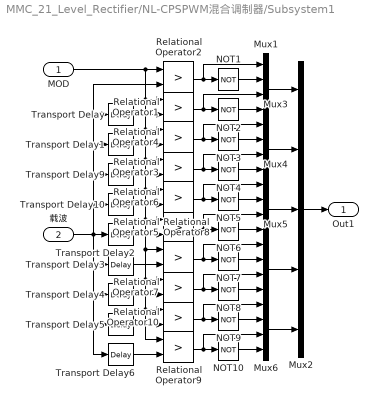
== system MMC_21_Level_Rectifier/NL-CPSPWM混合调制器/Subsystem1 ==
  MOD : Inport
  载波 : Inport  Port=2
  Mux{1,3..6} (5 alike) : Mux
  Mux2 : Mux  Inputs=5
  NOT{1..10} (10 alike) : Logic  Operator=NOT  IconShape=distinctive  AllPortsSameDT=off  OutDataTypeStr=boolean
  Relational Operator{1..10} (10 alike) : RelationalOperator  Operator=>  OutDataTypeStr=boolean  InputSameDT=off
  Transport Delay : TransportDelay  DelayTime=1/800/10
  Transport Delay1 : TransportDelay  DelayTime=2/800/10
  Transport Delay10 : TransportDelay  DelayTime=4/800/10
  Transport Delay2 : TransportDelay  DelayTime=5/800/10
  Transport Delay3 : TransportDelay  DelayTime=6/800/10
  Transport Delay4 : TransportDelay  DelayTime=7/800/10
  Transport Delay5 : TransportDelay  DelayTime=8/800/10
  Transport Delay6 : TransportDelay  DelayTime=9/800/10
  Transport Delay9 : TransportDelay  DelayTime=3/800/10
  Out1 : Outport
  wires:
  MOD/1 -> Relational Operator2/1, Relational Operator1/1, Relational Operator4/1, Relational Operator3/1, Relational Operator6/1, Relational Operator5/1, Relational Operator8/1, Relational Operator7/1, Relational Operator10/1, Relational Operator9/1
  Transport Delay6/1 -> Relational Operator9/2
  Transport Delay5/1 -> Relational Operator10/2
  Transport Delay4/1 -> Relational Operator7/2
  Transport Delay3/1 -> Relational Operator8/2
  Transport Delay2/1 -> Relational Operator5/2
  Transport Delay/1 -> Relational Operator1/2
  Relational Operator10/1 -> Mux6/1, NOT9/1
  NOT9/1 -> Mux6/2
  Relational Operator9/1 -> Mux6/3, NOT10/1
  NOT10/1 -> Mux6/4
  Mux6/1 -> Mux2/5
  Relational Operator6/1 -> Mux4/1, NOT5/1
  NOT5/1 -> Mux4/2
  Relational Operator5/1 -> Mux4/3, NOT6/1
  NOT6/1 -> Mux4/4
  Mux4/1 -> Mux2/3
  Mux5/1 -> Mux2/4
  NOT8/1 -> Mux5/4
  Relational Operator7/1 -> NOT8/1, Mux5/3
  NOT7/1 -> Mux5/2
  Relational Operator8/1 -> NOT7/1, Mux5/1
  Relational Operator4/1 -> Mux3/1, NOT3/1
  NOT3/1 -> Mux3/2
  Relational Operator3/1 -> Mux3/3, NOT4/1
  NOT4/1 -> Mux3/4
  Mux3/1 -> Mux2/2
  Mux1/1 -> Mux2/1
  NOT2/1 -> Mux1/4
  Relational Operator1/1 -> NOT2/1, Mux1/3
  NOT1/1 -> Mux1/2
  Relational Operator2/1 -> NOT1/1, Mux1/1
  Transport Delay10/1 -> Relational Operator6/2
  Mux2/1 -> Out1/1
  Transport Delay9/1 -> Relational Operator3/2
  Transport Delay1/1 -> Relational Operator4/2
  载波/1 -> Transport Delay3/1, Transport Delay4/1, Transport Delay5/1, Transport Delay6/1, Transport Delay10/1, Transport Delay9/1, Transport Delay1/1, Transport Delay/1, Relational Operator2/2, Transport Delay2/1

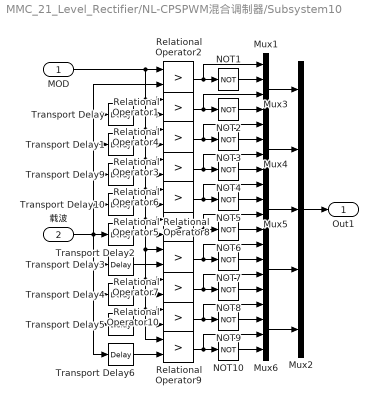
== system MMC_21_Level_Rectifier/NL-CPSPWM混合调制器/Subsystem10 ==
  MOD : Inport
  载波 : Inport  Port=2
  Mux{1,3..6} (5 alike) : Mux
  Mux2 : Mux  Inputs=5
  NOT{1..10} (10 alike) : Logic  Operator=NOT  IconShape=distinctive  AllPortsSameDT=off  OutDataTypeStr=boolean
  Relational Operator{1..10} (10 alike) : RelationalOperator  Operator=>  OutDataTypeStr=boolean  InputSameDT=off
  Transport Delay : TransportDelay  DelayTime=1/800/10
  Transport Delay1 : TransportDelay  DelayTime=2/800/10
  Transport Delay10 : TransportDelay  DelayTime=4/800/10
  Transport Delay2 : TransportDelay  DelayTime=5/800/10
  Transport Delay3 : TransportDelay  DelayTime=6/800/10
  Transport Delay4 : TransportDelay  DelayTime=7/800/10
  Transport Delay5 : TransportDelay  DelayTime=8/800/10
  Transport Delay6 : TransportDelay  DelayTime=9/800/10
  Transport Delay9 : TransportDelay  DelayTime=3/800/10
  Out1 : Outport
  wires:
  载波/1 -> Transport Delay2/1, Relational Operator2/2, Transport Delay/1, Transport Delay1/1, Transport Delay9/1, Transport Delay10/1, Transport Delay6/1, Transport Delay5/1, Transport Delay4/1, Transport Delay3/1
  Transport Delay1/1 -> Relational Operator4/2
  Transport Delay9/1 -> Relational Operator3/2
  Mux2/1 -> Out1/1
  Transport Delay10/1 -> Relational Operator6/2
  Relational Operator2/1 -> Mux1/1, NOT1/1
  NOT1/1 -> Mux1/2
  Relational Operator1/1 -> Mux1/3, NOT2/1
  NOT2/1 -> Mux1/4
  Mux1/1 -> Mux2/1
  Mux3/1 -> Mux2/2
  NOT4/1 -> Mux3/4
  Relational Operator3/1 -> NOT4/1, Mux3/3
  NOT3/1 -> Mux3/2
  Relational Operator4/1 -> NOT3/1, Mux3/1
  Relational Operator8/1 -> Mux5/1, NOT7/1
  NOT7/1 -> Mux5/2
  Relational Operator7/1 -> Mux5/3, NOT8/1
  NOT8/1 -> Mux5/4
  Mux5/1 -> Mux2/4
  Mux4/1 -> Mux2/3
  NOT6/1 -> Mux4/4
  Relational Operator5/1 -> NOT6/1, Mux4/3
  NOT5/1 -> Mux4/2
  Relational Operator6/1 -> NOT5/1, Mux4/1
  Mux6/1 -> Mux2/5
  NOT10/1 -> Mux6/4
  Relational Operator9/1 -> NOT10/1, Mux6/3
  NOT9/1 -> Mux6/2
  Relational Operator10/1 -> NOT9/1, Mux6/1
  Transport Delay/1 -> Relational Operator1/2
  Transport Delay2/1 -> Relational Operator5/2
  Transport Delay3/1 -> Relational Operator8/2
  Transport Delay4/1 -> Relational Operator7/2
  Transport Delay5/1 -> Relational Operator10/2
  Transport Delay6/1 -> Relational Operator9/2
  MOD/1 -> Relational Operator9/1, Relational Operator10/1, Relational Operator7/1, Relational Operator8/1, Relational Operator5/1, Relational Operator6/1, Relational Operator3/1, Relational Operator4/1, Relational Operator1/1, Relational Operator2/1

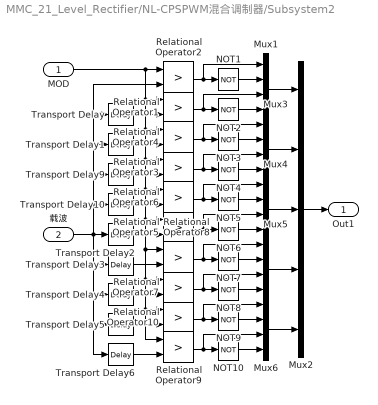
== system MMC_21_Level_Rectifier/NL-CPSPWM混合调制器/Subsystem2 ==
  MOD : Inport
  载波 : Inport  Port=2
  Mux{1,3..6} (5 alike) : Mux
  Mux2 : Mux  Inputs=5
  NOT{1..10} (10 alike) : Logic  Operator=NOT  IconShape=distinctive  AllPortsSameDT=off  OutDataTypeStr=boolean
  Relational Operator{1..10} (10 alike) : RelationalOperator  Operator=>  OutDataTypeStr=boolean  InputSameDT=off
  Transport Delay : TransportDelay  DelayTime=1/800/10
  Transport Delay1 : TransportDelay  DelayTime=2/800/10
  Transport Delay10 : TransportDelay  DelayTime=4/800/10
  Transport Delay2 : TransportDelay  DelayTime=5/800/10
  Transport Delay3 : TransportDelay  DelayTime=6/800/10
  Transport Delay4 : TransportDelay  DelayTime=7/800/10
  Transport Delay5 : TransportDelay  DelayTime=8/800/10
  Transport Delay6 : TransportDelay  DelayTime=9/800/10
  Transport Delay9 : TransportDelay  DelayTime=3/800/10
  Out1 : Outport
  wires:
  载波/1 -> Transport Delay2/1, Relational Operator2/2, Transport Delay/1, Transport Delay1/1, Transport Delay9/1, Transport Delay10/1, Transport Delay6/1, Transport Delay5/1, Transport Delay4/1, Transport Delay3/1
  Transport Delay1/1 -> Relational Operator4/2
  Transport Delay9/1 -> Relational Operator3/2
  Mux2/1 -> Out1/1
  Transport Delay10/1 -> Relational Operator6/2
  Relational Operator2/1 -> Mux1/1, NOT1/1
  NOT1/1 -> Mux1/2
  Relational Operator1/1 -> Mux1/3, NOT2/1
  NOT2/1 -> Mux1/4
  Mux1/1 -> Mux2/1
  Mux3/1 -> Mux2/2
  NOT4/1 -> Mux3/4
  Relational Operator3/1 -> NOT4/1, Mux3/3
  NOT3/1 -> Mux3/2
  Relational Operator4/1 -> NOT3/1, Mux3/1
  Relational Operator8/1 -> Mux5/1, NOT7/1
  NOT7/1 -> Mux5/2
  Relational Operator7/1 -> Mux5/3, NOT8/1
  NOT8/1 -> Mux5/4
  Mux5/1 -> Mux2/4
  Mux4/1 -> Mux2/3
  NOT6/1 -> Mux4/4
  Relational Operator5/1 -> NOT6/1, Mux4/3
  NOT5/1 -> Mux4/2
  Relational Operator6/1 -> NOT5/1, Mux4/1
  Mux6/1 -> Mux2/5
  NOT10/1 -> Mux6/4
  Relational Operator9/1 -> NOT10/1, Mux6/3
  NOT9/1 -> Mux6/2
  Relational Operator10/1 -> NOT9/1, Mux6/1
  Transport Delay/1 -> Relational Operator1/2
  Transport Delay2/1 -> Relational Operator5/2
  Transport Delay3/1 -> Relational Operator8/2
  Transport Delay4/1 -> Relational Operator7/2
  Transport Delay5/1 -> Relational Operator10/2
  Transport Delay6/1 -> Relational Operator9/2
  MOD/1 -> Relational Operator9/1, Relational Operator10/1, Relational Operator7/1, Relational Operator8/1, Relational Operator5/1, Relational Operator6/1, Relational Operator3/1, Relational Operator4/1, Relational Operator1/1, Relational Operator2/1

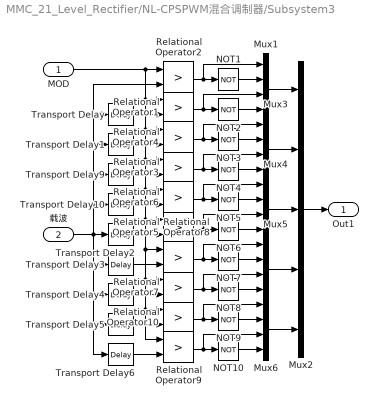
== system MMC_21_Level_Rectifier/NL-CPSPWM混合调制器/Subsystem3 ==
  MOD : Inport
  载波 : Inport  Port=2
  Mux{1,3..6} (5 alike) : Mux
  Mux2 : Mux  Inputs=5
  NOT{1..10} (10 alike) : Logic  Operator=NOT  IconShape=distinctive  AllPortsSameDT=off  OutDataTypeStr=boolean
  Relational Operator{1..10} (10 alike) : RelationalOperator  Operator=>  OutDataTypeStr=boolean  InputSameDT=off
  Transport Delay : TransportDelay  DelayTime=1/800/10
  Transport Delay1 : TransportDelay  DelayTime=2/800/10
  Transport Delay10 : TransportDelay  DelayTime=4/800/10
  Transport Delay2 : TransportDelay  DelayTime=5/800/10
  Transport Delay3 : TransportDelay  DelayTime=6/800/10
  Transport Delay4 : TransportDelay  DelayTime=7/800/10
  Transport Delay5 : TransportDelay  DelayTime=8/800/10
  Transport Delay6 : TransportDelay  DelayTime=9/800/10
  Transport Delay9 : TransportDelay  DelayTime=3/800/10
  Out1 : Outport
  wires:
  MOD/1 -> Relational Operator2/1, Relational Operator1/1, Relational Operator4/1, Relational Operator3/1, Relational Operator6/1, Relational Operator5/1, Relational Operator8/1, Relational Operator7/1, Relational Operator10/1, Relational Operator9/1
  Transport Delay6/1 -> Relational Operator9/2
  Transport Delay5/1 -> Relational Operator10/2
  Transport Delay4/1 -> Relational Operator7/2
  Transport Delay3/1 -> Relational Operator8/2
  Transport Delay2/1 -> Relational Operator5/2
  Transport Delay/1 -> Relational Operator1/2
  Relational Operator10/1 -> Mux6/1, NOT9/1
  NOT9/1 -> Mux6/2
  Relational Operator9/1 -> Mux6/3, NOT10/1
  NOT10/1 -> Mux6/4
  Mux6/1 -> Mux2/5
  Relational Operator6/1 -> Mux4/1, NOT5/1
  NOT5/1 -> Mux4/2
  Relational Operator5/1 -> Mux4/3, NOT6/1
  NOT6/1 -> Mux4/4
  Mux4/1 -> Mux2/3
  Mux5/1 -> Mux2/4
  NOT8/1 -> Mux5/4
  Relational Operator7/1 -> NOT8/1, Mux5/3
  NOT7/1 -> Mux5/2
  Relational Operator8/1 -> NOT7/1, Mux5/1
  Relational Operator4/1 -> Mux3/1, NOT3/1
  NOT3/1 -> Mux3/2
  Relational Operator3/1 -> Mux3/3, NOT4/1
  NOT4/1 -> Mux3/4
  Mux3/1 -> Mux2/2
  Mux1/1 -> Mux2/1
  NOT2/1 -> Mux1/4
  Relational Operator1/1 -> NOT2/1, Mux1/3
  NOT1/1 -> Mux1/2
  Relational Operator2/1 -> NOT1/1, Mux1/1
  Transport Delay10/1 -> Relational Operator6/2
  Mux2/1 -> Out1/1
  Transport Delay9/1 -> Relational Operator3/2
  Transport Delay1/1 -> Relational Operator4/2
  载波/1 -> Transport Delay3/1, Transport Delay4/1, Transport Delay5/1, Transport Delay6/1, Transport Delay10/1, Transport Delay9/1, Transport Delay1/1, Transport Delay/1, Relational Operator2/2, Transport Delay2/1

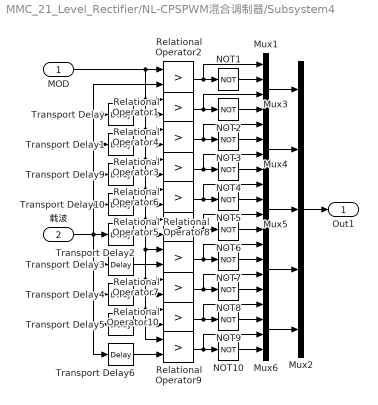
== system MMC_21_Level_Rectifier/NL-CPSPWM混合调制器/Subsystem4 ==
  MOD : Inport
  载波 : Inport  Port=2
  Mux{1,3..6} (5 alike) : Mux
  Mux2 : Mux  Inputs=5
  NOT{1..10} (10 alike) : Logic  Operator=NOT  IconShape=distinctive  AllPortsSameDT=off  OutDataTypeStr=boolean
  Relational Operator{1..10} (10 alike) : RelationalOperator  Operator=>  OutDataTypeStr=boolean  InputSameDT=off
  Transport Delay : TransportDelay  DelayTime=1/800/10
  Transport Delay1 : TransportDelay  DelayTime=2/800/10
  Transport Delay10 : TransportDelay  DelayTime=4/800/10
  Transport Delay2 : TransportDelay  DelayTime=5/800/10
  Transport Delay3 : TransportDelay  DelayTime=6/800/10
  Transport Delay4 : TransportDelay  DelayTime=7/800/10
  Transport Delay5 : TransportDelay  DelayTime=8/800/10
  Transport Delay6 : TransportDelay  DelayTime=9/800/10
  Transport Delay9 : TransportDelay  DelayTime=3/800/10
  Out1 : Outport
  wires:
  载波/1 -> Transport Delay2/1, Relational Operator2/2, Transport Delay/1, Transport Delay1/1, Transport Delay9/1, Transport Delay10/1, Transport Delay6/1, Transport Delay5/1, Transport Delay4/1, Transport Delay3/1
  Transport Delay1/1 -> Relational Operator4/2
  Transport Delay9/1 -> Relational Operator3/2
  Mux2/1 -> Out1/1
  Transport Delay10/1 -> Relational Operator6/2
  Relational Operator2/1 -> Mux1/1, NOT1/1
  NOT1/1 -> Mux1/2
  Relational Operator1/1 -> Mux1/3, NOT2/1
  NOT2/1 -> Mux1/4
  Mux1/1 -> Mux2/1
  Mux3/1 -> Mux2/2
  NOT4/1 -> Mux3/4
  Relational Operator3/1 -> NOT4/1, Mux3/3
  NOT3/1 -> Mux3/2
  Relational Operator4/1 -> NOT3/1, Mux3/1
  Relational Operator8/1 -> Mux5/1, NOT7/1
  NOT7/1 -> Mux5/2
  Relational Operator7/1 -> Mux5/3, NOT8/1
  NOT8/1 -> Mux5/4
  Mux5/1 -> Mux2/4
  Mux4/1 -> Mux2/3
  NOT6/1 -> Mux4/4
  Relational Operator5/1 -> NOT6/1, Mux4/3
  NOT5/1 -> Mux4/2
  Relational Operator6/1 -> NOT5/1, Mux4/1
  Mux6/1 -> Mux2/5
  NOT10/1 -> Mux6/4
  Relational Operator9/1 -> NOT10/1, Mux6/3
  NOT9/1 -> Mux6/2
  Relational Operator10/1 -> NOT9/1, Mux6/1
  Transport Delay/1 -> Relational Operator1/2
  Transport Delay2/1 -> Relational Operator5/2
  Transport Delay3/1 -> Relational Operator8/2
  Transport Delay4/1 -> Relational Operator7/2
  Transport Delay5/1 -> Relational Operator10/2
  Transport Delay6/1 -> Relational Operator9/2
  MOD/1 -> Relational Operator9/1, Relational Operator10/1, Relational Operator7/1, Relational Operator8/1, Relational Operator5/1, Relational Operator6/1, Relational Operator3/1, Relational Operator4/1, Relational Operator1/1, Relational Operator2/1

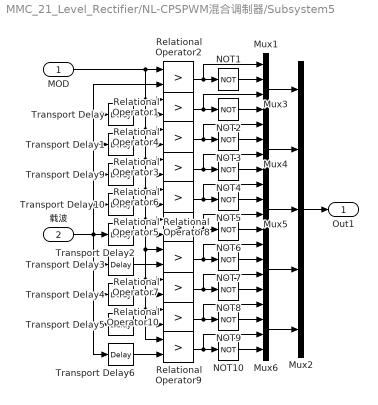
== system MMC_21_Level_Rectifier/NL-CPSPWM混合调制器/Subsystem5 ==
  MOD : Inport
  载波 : Inport  Port=2
  Mux{1,3..6} (5 alike) : Mux
  Mux2 : Mux  Inputs=5
  NOT{1..10} (10 alike) : Logic  Operator=NOT  IconShape=distinctive  AllPortsSameDT=off  OutDataTypeStr=boolean
  Relational Operator{1..10} (10 alike) : RelationalOperator  Operator=>  OutDataTypeStr=boolean  InputSameDT=off
  Transport Delay : TransportDelay  DelayTime=1/800/10
  Transport Delay1 : TransportDelay  DelayTime=2/800/10
  Transport Delay10 : TransportDelay  DelayTime=4/800/10
  Transport Delay2 : TransportDelay  DelayTime=5/800/10
  Transport Delay3 : TransportDelay  DelayTime=6/800/10
  Transport Delay4 : TransportDelay  DelayTime=7/800/10
  Transport Delay5 : TransportDelay  DelayTime=8/800/10
  Transport Delay6 : TransportDelay  DelayTime=9/800/10
  Transport Delay9 : TransportDelay  DelayTime=3/800/10
  Out1 : Outport
  wires:
  MOD/1 -> Relational Operator2/1, Relational Operator1/1, Relational Operator4/1, Relational Operator3/1, Relational Operator6/1, Relational Operator5/1, Relational Operator8/1, Relational Operator7/1, Relational Operator10/1, Relational Operator9/1
  Transport Delay6/1 -> Relational Operator9/2
  Transport Delay5/1 -> Relational Operator10/2
  Transport Delay4/1 -> Relational Operator7/2
  Transport Delay3/1 -> Relational Operator8/2
  Transport Delay2/1 -> Relational Operator5/2
  Transport Delay/1 -> Relational Operator1/2
  Relational Operator10/1 -> Mux6/1, NOT9/1
  NOT9/1 -> Mux6/2
  Relational Operator9/1 -> Mux6/3, NOT10/1
  NOT10/1 -> Mux6/4
  Mux6/1 -> Mux2/5
  Relational Operator6/1 -> Mux4/1, NOT5/1
  NOT5/1 -> Mux4/2
  Relational Operator5/1 -> Mux4/3, NOT6/1
  NOT6/1 -> Mux4/4
  Mux4/1 -> Mux2/3
  Mux5/1 -> Mux2/4
  NOT8/1 -> Mux5/4
  Relational Operator7/1 -> NOT8/1, Mux5/3
  NOT7/1 -> Mux5/2
  Relational Operator8/1 -> NOT7/1, Mux5/1
  Relational Operator4/1 -> Mux3/1, NOT3/1
  NOT3/1 -> Mux3/2
  Relational Operator3/1 -> Mux3/3, NOT4/1
  NOT4/1 -> Mux3/4
  Mux3/1 -> Mux2/2
  Mux1/1 -> Mux2/1
  NOT2/1 -> Mux1/4
  Relational Operator1/1 -> NOT2/1, Mux1/3
  NOT1/1 -> Mux1/2
  Relational Operator2/1 -> NOT1/1, Mux1/1
  Transport Delay10/1 -> Relational Operator6/2
  Mux2/1 -> Out1/1
  Transport Delay9/1 -> Relational Operator3/2
  Transport Delay1/1 -> Relational Operator4/2
  载波/1 -> Transport Delay3/1, Transport Delay4/1, Transport Delay5/1, Transport Delay6/1, Transport Delay10/1, Transport Delay9/1, Transport Delay1/1, Transport Delay/1, Relational Operator2/2, Transport Delay2/1

== system MMC_21_Level_Rectifier/PIR均压和环流抑制器/PIR ==
  err : Inport
  Integrator : Integrator
  Kp : Gain  Gain=Kp
  Kr : Gain  Gain=Kr
  Saturation : Saturate  UpperLimit=Upper  LowerLimit=Lower
  Sum3 : Sum  Inputs=+++
  Transfer Fcn : TransferFcn  Numerator=[2*Wc 0]  Denominator=[1 2*Wc 628^2]
  ref : Outport
  wires:
  Kr/1 -> Transfer Fcn/1
  Saturation/1 -> ref/1
  Sum3/1 -> Saturation/1
  err/1 -> Kr/1, Kp/1
  Integrator/1 -> Sum3/1
  Kp/1 -> Integrator/1, Sum3/2
  Transfer Fcn/1 -> Sum3/3

== system MMC_21_Level_Rectifier/PIR均压和环流抑制器/PIR1 ==
  err : Inport
  Integrator : Integrator
  Kp : Gain  Gain=Kp
  Kr : Gain  Gain=Kr
  Saturation : Saturate  UpperLimit=Upper  LowerLimit=Lower
  Sum3 : Sum  Inputs=+++
  Transfer Fcn : TransferFcn  Numerator=[2*Wc 0]  Denominator=[1 2*Wc 628^2]
  ref : Outport
  wires:
  Transfer Fcn/1 -> Sum3/3
  Kp/1 -> Sum3/2, Integrator/1
  Integrator/1 -> Sum3/1
  err/1 -> Kp/1, Kr/1
  Sum3/1 -> Saturation/1
  Saturation/1 -> ref/1
  Kr/1 -> Transfer Fcn/1

== system MMC_21_Level_Rectifier/PIR均压和环流抑制器/PIR2 ==
  err : Inport
  Integrator : Integrator
  Kp : Gain  Gain=Kp
  Kr : Gain  Gain=Kr
  Saturation : Saturate  UpperLimit=Upper  LowerLimit=Lower
  Sum3 : Sum  Inputs=+++
  Transfer Fcn : TransferFcn  Numerator=[2*Wc 0]  Denominator=[1 2*Wc 628^2]
  ref : Outport
  wires:
  Kr/1 -> Transfer Fcn/1
  Saturation/1 -> ref/1
  Sum3/1 -> Saturation/1
  err/1 -> Kr/1, Kp/1
  Integrator/1 -> Sum3/1
  Kp/1 -> Integrator/1, Sum3/2
  Transfer Fcn/1 -> Sum3/3

== system MMC_21_Level_Rectifier/PIR均压和环流抑制器/PIR3 ==
  err : Inport
  Integrator : Integrator
  Kp : Gain  Gain=Kp
  Kr : Gain  Gain=Kr
  Saturation : Saturate  UpperLimit=Upper  LowerLimit=Lower
  Sum3 : Sum  Inputs=+++
  Transfer Fcn : TransferFcn  Numerator=[2*Wc 0]  Denominator=[1 2*Wc 628^2]
  ref : Outport
  wires:
  Transfer Fcn/1 -> Sum3/3
  Kp/1 -> Sum3/2, Integrator/1
  Integrator/1 -> Sum3/1
  err/1 -> Kp/1, Kr/1
  Sum3/1 -> Saturation/1
  Saturation/1 -> ref/1
  Kr/1 -> Transfer Fcn/1

== system MMC_21_Level_Rectifier/PIR均压和环流抑制器/PIR4 ==
  err : Inport
  Integrator : Integrator
  Kp : Gain  Gain=Kp
  Kr : Gain  Gain=Kr
  Saturation : Saturate  UpperLimit=Upper  LowerLimit=Lower
  Sum3 : Sum  Inputs=+++
  Transfer Fcn : TransferFcn  Numerator=[2*Wc 0]  Denominator=[1 2*Wc 628^2]
  ref : Outport
  wires:
  Kr/1 -> Transfer Fcn/1
  Saturation/1 -> ref/1
  Sum3/1 -> Saturation/1
  err/1 -> Kr/1, Kp/1
  Integrator/1 -> Sum3/1
  Kp/1 -> Integrator/1, Sum3/2
  Transfer Fcn/1 -> Sum3/3

== system MMC_21_Level_Rectifier/PIR均压和环流抑制器/PIR5 ==
  err : Inport
  Integrator : Integrator
  Kp : Gain  Gain=Kp
  Kr : Gain  Gain=Kr
  Saturation : Saturate  UpperLimit=Upper  LowerLimit=Lower
  Sum3 : Sum  Inputs=+++
  Transfer Fcn : TransferFcn  Numerator=[2*Wc 0]  Denominator=[1 2*Wc 628^2]
  ref : Outport
  wires:
  Transfer Fcn/1 -> Sum3/3
  Kp/1 -> Sum3/2, Integrator/1
  Integrator/1 -> Sum3/1
  err/1 -> Kp/1, Kr/1
  Sum3/1 -> Saturation/1
  Saturation/1 -> ref/1
  Kr/1 -> Transfer Fcn/1
